simulink model "DDMR_OpenLoop"  (R2024b)
settings: Solver=VariableStepAuto  StartTime=0.0  StopTime=15  RelTol=1e-3
values from neighbouring files (symbols this model uses):
  L = 0.2    [LQR.m]    (also in Track.m; Track2.m)
  R = 0.05    [LQR.m]    (also in Track.m; Track2.m)
libraries: robotmobilelib x1
settings Model: Creator=moham  LastModifiedBy=moham

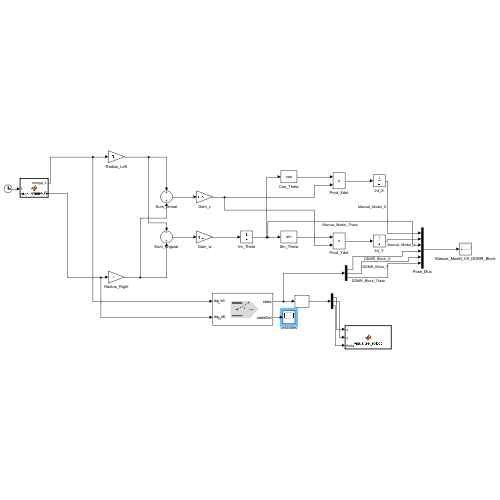
[thumbnail: Simulink's stored preview of the top-level diagram]
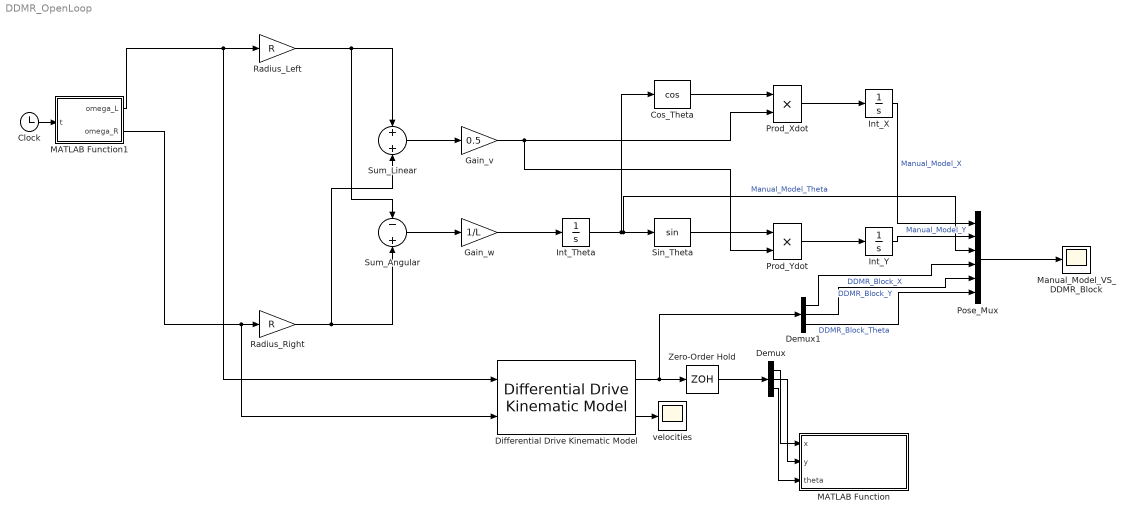
== system DDMR_OpenLoop ==
  Clock : Clock
  Cos_Theta : Trigonometry  Operator=cos
  Demux : Demux  Outputs=3
  Demux1 : Demux  Outputs=3
  Differential Drive Kinematic Model : robotmobilelib/Differential Drive Kinematic Model  VehicleInputs=Wheel Speeds  WheelRadius=0.05  WheelSpeedRange=[-inf inf]  TrackWidth=0.2  InitialState=[0; 0; 0]  SimulateUsing=Interpreted execution
  Gain_v : Gain  Gain=0.5
  Gain_w : Gain  Gain=1/L
  Int_Theta : Integrator
  Int_X : Integrator
  Int_Y : Integrator
  MATLAB Function : MATLAB Function  TreatAsAtomicUnit=on
  MATLAB Function1 : MATLAB Function  TreatAsAtomicUnit=on
  Manual_Model_VS_DDMR_Block : Scope
  Pose_Mux : Mux  Inputs=6
  Prod_Xdot : Product
  Prod_Ydot : Product
  Radius_Left : Gain  Gain=R
  Radius_Right : Gain  Gain=R
  Sin_Theta : Trigonometry
  Sum_Angular : Sum  Inputs=-+
  Sum_Linear : Sum
  Zero-Order Hold : ZeroOrderHold  SampleTime=0.05
  velocities : Scope
  wires:
  MATLAB Function1/1(omega_L) -> Differential Drive Kinematic Model/1, Radius_Left/1
  Differential Drive Kinematic Model/1 -> Demux1/1, Zero-Order Hold/1
  Demux/1 -> MATLAB Function/1(x)
  MATLAB Function1/2(omega_R) -> Differential Drive Kinematic Model/2, Radius_Right/1
  Prod_Ydot/1 -> Int_Y/1
  Int_Theta/1 -> Pose_Mux/3, Sin_Theta/1, Cos_Theta/1  "Manual_Model_Theta"
  Differential Drive Kinematic Model/2 -> velocities/1
  Int_Y/1 -> Pose_Mux/2  "Manual_Model_Y"
  Int_X/1 -> Pose_Mux/1  "Manual_Model_X"
  Cos_Theta/1 -> Prod_Xdot/1
  Gain_v/1 -> Prod_Xdot/2, Prod_Ydot/2
  Sin_Theta/1 -> Prod_Ydot/1
  Prod_Xdot/1 -> Int_X/1
  Demux/2 -> MATLAB Function/2(y)
  Gain_w/1 -> Int_Theta/1
  Radius_Left/1 -> Sum_Linear/1, Sum_Angular/1
  Sum_Angular/1 -> Gain_w/1
  Radius_Right/1 -> Sum_Linear/2, Sum_Angular/2
  Pose_Mux/1 -> Manual_Model_VS_DDMR_Block/1
  Sum_Linear/1 -> Gain_v/1
  Demux/3 -> MATLAB Function/3(theta)
  Zero-Order Hold/1 -> Demux/1
  Clock/1 -> MATLAB Function1/1(t)
  Demux1/1 -> Pose_Mux/4  "DDMR_Block_X"
  Demux1/2 -> Pose_Mux/5  "DDMR_Block_Y"
  Demux1/3 -> Pose_Mux/6  "DDMR_Block_Theta"

== matlab function DDMR_OpenLoop/MATLAB Function ==
  data: x input; y input; theta input
function visualize_robot(x, y, theta)
    % Tell Simulink to execute plotting functions in MATLAB, not as C code
    coder.extrinsic('figure', 'plot', 'set', 'drawnow', 'axis', 'grid', 'hold', 'isvalid');
    
    % Declare persistent variables
    persistent fig hCircle hLine
    
    r = 0.5; % Radius of the robot
    line_length = 2 * r; % How far the heading line extends
    
    % Safely check if the figure is unassigned
    if isempty(fig)
        % First time initialization
        fig = figure('Name', 'Robot Pose Visualization');
        hold on; 
        grid on; 
        axis equal;
        axis([-15 15 -15 15]); 
        
        th = linspace(0, 2*pi, 50);
        hCircle = plot(x + r*cos(th), y + r*sin(th), 'b-', 'LineWidth', 1.5);
        
        % Multiply by line_length instead of r
        hLine = plot([x, x + line_length*cos(theta)], [y, y + line_length*sin(theta)], 'r-', 'LineWidth', 2);
        
    % Safely check if the figure was closed by the user mid-simulation
    elseif ~isvalid(fig)
        % Re-initialize
        fig = figure('Name', 'Robot Pose Visualization');
        hold on; 
        grid on; 
        axis equal;
        axis([-15 15 -15 15]); 
        
        th = linspace(0, 2*pi, 50);
        hCircle = plot(x + r*cos(th), y + r*sin(th), 'b-', 'LineWidth', 1.5);
        
        % Multiply by line_length instead of r
        hLine = plot([x, x + line_length*cos(theta)], [y, y + line_length*sin(theta)], 'r-', 'LineWidth', 2);
        
    else
        % Update the existing plot objects
        th = linspace(0, 2*pi, 50);
        set(hCircle, 'XData', x + r*cos(th), 'YData', y + r*sin(th));
        
        % Multiply by line_length instead of r
        set(hLine, 'XData', [x, x + line_length*cos(theta)], 'YData', [y, y + line_length*sin(theta)]);
    end
    
    drawnow limitrate;
end

== matlab function DDMR_OpenLoop/MATLAB Function1 ==
  data: t input; omega_L output; omega_R output
function [omega_L, omega_R] = motor_commands(t)

    % Interval 1: From 0 to 4 seconds -> Drive straight
    if t < 4.0
        omega_L = 6;
        omega_R = 6;
        
    % Interval 2: From 4 to 8 seconds -> Turn smoothly to the LEFT
    elseif t < 8.0
        omega_L = 2;
        omega_R = 6;
        
    % Interval 3: From 8 to 11 seconds -> Drive straight again
    elseif t < 11.0
        omega_L = 3;
        omega_R = 3;
        
    % Interval 4: From 11 to 14 seconds -> Spin in place
    elseif t < 14.0
        omega_L = -4;
        omega_R = 4;
        
    % Interval 5: 14 to 15 seconds -> Stop
    else
        omega_L = 0;
        omega_R = 0;
    end

end
